simulink model "AFC_FFNN_trainbfg_60_60_60_Nor_July_15_RepFast"  (R2021a)
settings: Solver=ode15s  StartTime=0.0  StopTime=T  MaxStep=.01  RelTol=1e-3
undefined symbols (not defined in the file): AF_sensor_tol, fault_time, fuel_inj_tol, kappa_tol, MAF_sensor_tol, patch_sig, pump_tol, safe_patch_sig, sw, tau_ww_tol, x_gain, x_offset, y_gain, y_offset
libraries: neural x185, simulink x3
(part 8 of 8)

== system AFC_FFNN_trainbfg_60_60_60_Nor_July_15_RepFast/Air Fuel Control Model 1/Feed-Forward Neural Network/Layer 4/Delays 1 ==
  "p{4}" : Inport  PortDimensions=60
      mask Display: e = 0.06;c1 = [120 230 180]/255;c2 = ([120 230 180]+0)/(256+128);c3 = ([120 230 180]+128)/(256+128);patch([0 1 1 0],[0 0 1 1],c1);patch([0 1 1 1-e 1-e 0+e],[0 0 1 1-e 0+e 0+e],c2);patch([0 0 1 1-e 0+e 0+e],[0 1 1 1-e 1-e 0+e],c3);plot([0 1 1 0 0],[0 0 1 1 0]);
  mux : Mux  Inputs=1
      mask Display: e = 0.06;c1 = [120 150 230]/255;c2 = ([120 150 230]+0)/383;c3 = ([120 150 230]+128)/383;patch([0 1 1 0],[0 0 1 1],c1);patch([0 1 1 1-e 1-e 0+e],[0 0 1 1-e 0+e 0+e],c2);patch([0 0 1 1-e 0+e 0+e],[0 1 1 1-e 1-e 0+e],c3);plot([0 1 1 0 0],[0 0 1 1 0]);disp('Mux')
  "pd{4,3}" : Outport
      mask Display: e = 0.06;c1 = [120 230 180]/255;c2 = ([120 230 180]+0)/(256+128);c3 = ([120 230 180]+128)/(256+128);patch([0 1 1 0],[0 0 1 1],c1);patch([0 1 1 1-e 1-e 0+e],[0 0 1 1-e 0+e 0+e],c2);patch([0 0 1 1-e 0+e 0+e],[0 1 1 1-e 1-e 0+e],c3);plot([0 1 1 0 0],[0 0 1 1 0]);
  wires:
  mux/1 -> "pd{4,3}"/1
  "p{4}"/1 -> mux/1

== system AFC_FFNN_trainbfg_60_60_60_Nor_July_15_RepFast/Air Fuel Control Model 1/Feed-Forward Neural Network/Layer 4/LW{4,3} ==
  "ad{4,3}" : Inport  PortDimensions=60
      mask Display: e = 0.06;c1 = [120 230 180]/255;c2 = ([120 230 180]+0)/(256+128);c3 = ([120 230 180]+128)/(256+128);patch([0 1 1 0],[0 0 1 1],c1);patch([0 1 1 1-e 1-e 0+e],[0 0 1 1-e 0+e 0+e],c2);patch([0 0 1 1-e 0+e 0+e],[0 1 1 1-e 1-e 0+e],c3);plot([0 1 1 0 0],[0 0 1 1 0]);
  "IW{4,3}(1,:)'" : Constant  Value=[0.49973643041457904701019288040697574615478515625;-0.447188171023051028729611289236345328390598297119140625;0.040497996394893660820901715169384260661900043487548828125;-0.176479086096453519072468907324946485459804534912109375;0.1943195232390433624392045430795405991375446319580078125;0.59406039211729133597827967605553567409515380859375;0.7167302436758060668609005006146617233753204345703125;0.384317545677302307982614593129255808889865875244140625;-0.24279001302591385336171470044064335525035858154296875;0.364326547162041214367178554311976768076419830322265625;0.2174367282595285610913293794510536827147006988525390625;0.08296568831028237889224641321561648510396480560302734375;0.79717281232517256395198046448058448731899261474609375;0.374447070851066377006333141252980567514896392822265625;0.269943183076197357195269432850182056427001953125;0.0188649545720423160444223498188875964842736721038818359375;-0.0005834610340678283817161808855189519817940890789031982421875;0.50716938606579831105847233629901893436908721923828125;-0.76715047774135103342274533133604563772678375244140625;-0.6036524728182273147325531681417487561702728271484375;0.63687998063414419380734443620895035564899444580078125;-0.0215655028620936155270282341689380700699985027313232421875;0.49290504363119058695019703009165823459625244140625;-0.06161238971935496799847697957375203259289264678955078125;-0.31194488549520571485373920950223691761493682861328125;0.54895993281561639154375598081969656050205230712890625;0.046936862614446552000035950413803220726549625396728515625;0.2397725121438134265883235229921410791575908660888671875;-0.482047889813103702660868066232069395482540130615234375;-0.6758206679448297560242053805268369615077972412109375;0.258678439423680017750228898876230232417583465576171875;-0.299553924062803123007370231789536774158477783203125;-0.73455608446885645168578093944233842194080352783203125;-0.295746782395659046915881162931327708065509796142578125;-0.291379444911494422942865867298678494989871978759765625;0.226822015924426245714329297697986476123332977294921875;-0.051523894852851297165852173520761425606906414031982421875;0.1377887955024919841573449730276479385793209075927734375;0.69953656885165493850564644162659533321857452392578125;0.861111095922591385232180982711724936962127685546875;0.1740228009079731463781826050762902013957500457763671875;0.439993685352456254111785938221146352589130401611328125;-0.78236033510799651846667757126851938664913177490234375;0.118813788470795655971556925578624941408634185791015625;0.854455585586606058967618082533590495586395263671875;-0.074806684294961234282794748651213012635707855224609375;-0.4767576664614707748768296369235031306743621826171875;-0.128785107789830821634069479841855354607105255126953125;-0.60408819382140055420649105144548229873180389404296875;-0.139039078030579188460791328907362185418605804443359375;-0.0928188746857278867974372360549750737845897674560546875;-0.2412386425835751080359870002212119288742542266845703125;-0.461515637023861058363394249681732617318630218505859375;-0.6144162925897294069699228202807717025279998779296875;-0.11096968720173616684832040846231393516063690185546875;-0.2018914063361896271686646286980248987674713134765625;-0.2454512765649821959268450655144988559186458587646484375;-0.60738849309352394012506692888564430177211761474609375;0.312872638692257398762563980199047364294528961181640625;-1.0299379717984724624812997717526741325855255126953125]
      mask Display: e = 0.06;c1 = [120 150 230]/255;c2 = ([120 150 230]+0)/383;c3 = ([120 150 230]+128)/383;patch([0 1 1 0],[0 0 1 1],c1);patch([0 1 1 1-e 1-e 0+e],[0 0 1 1-e 0+e 0+e],c2);patch([0 0 1 1-e 0+e 0+e],[0 1 1 1-e 1-e 0+e],c3);plot([0 1 1 0 0],[0 0 1 1 0]);disp('weights');
  Mux : Mux  Inputs=1
      mask Display: e = 0.06;c1 = [120 150 230]/255;c2 = ([120 150 230]+0)/383;c3 = ([120 150 230]+128)/383;patch([0 1 1 0],[0 0 1 1],c1);patch([0 1 1 1-e 1-e 0+e],[0 0 1 1-e 0+e 0+e],c2);patch([0 0 1 1-e 0+e 0+e],[0 1 1 1-e 1-e 0+e],c3);plot([0 1 1 0 0],[0 0 1 1 0]);disp('Mux');
  dotprod1 : neural/Weight Functions/dotprod
  "lz{4,3}" : Outport
      mask Display: e = 0.06;c1 = [120 230 180]/255;c2 = ([120 230 180]+0)/(256+128);c3 = ([120 230 180]+128)/(256+128);patch([0 1 1 0],[0 0 1 1],c1);patch([0 1 1 1-e 1-e 0+e],[0 0 1 1-e 0+e 0+e],c2);patch([0 0 1 1-e 0+e 0+e],[0 1 1 1-e 1-e 0+e],c3);plot([0 1 1 0 0],[0 0 1 1 0]);
  wires:
  Mux/1 -> "lz{4,3}"/1
  dotprod1/1 -> Mux/1
  "ad{4,3}"/1 -> dotprod1/2
  "IW{4,3}(1,:)'"/1 -> dotprod1/1
